simulink model "Single_Tank_Model"  (R2026b)
settings: Solver=VariableStepAuto  StopTime=50
values from neighbouring files (symbols this model uses):
  A = 1    [run_simulation.m]
  c = 0.5    [run_simulation.m]
settings Model: Creator=gauravkeshava  LastModifiedBy=gauravkeshava

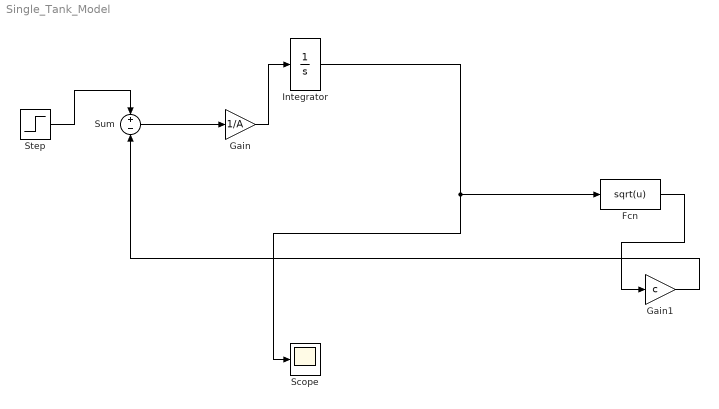
== system Single_Tank_Model ==
  Fcn : Fcn  Expr=sqrt(u)
  Gain : Gain  Gain=1/A
  Gain1 : Gain  Gain=c
  Integrator : Integrator  InitialCondition=0.25
  Scope : Scope
      settings: ActiveDisplayYMinimum=-0.21806585408171952  ActiveDisplayYMaximum=4.4625926867354764
  Step : Step  Time=0  SampleTime=0
  Sum : Sum  Inputs=+-
  wires:
  Step/1 -> Sum/1
  Sum/1 -> Gain/1
  Gain/1 -> Integrator/1
  Integrator/1 -> Scope/1, Fcn/1
  Fcn/1 -> Gain1/1
  Gain1/1 -> Sum/2
